simulink model "v2_2025_10_22_D1_chart_skeleton"  (R2025a)
settings: Solver=FixedStepAuto  StartTime=0.0  StopTime=10.0  FixedStep=1e-3  RelTol=1e-3  EnableMultiTasking=on
settings Model: ExtModeTrigDuration=5  Creator=zhang  LastModifiedBy=zhang
settings OptimizationCC: DefaultParameterBehavior=Inlined  EnhancedBackFolding=on  PassReuseOutputArgsAs=Individual arguments  ZeroExternalMemoryAtStartup=off  ZeroInternalMemoryAtStartup=off  MaxStackSize=64  OptimizeBlockOrder=speed  DifferentSizesBufferReuse=on  OptimizationCustomize=off  EfficientTunableParamExpr=on
settings DebuggingCC: ParameterTunabilityLossMsg=error
settings HardwareCC: ProdBitPerPointer=32.0  ProdBitPerSizeT=32.0  ProdBitPerPtrDiffT=32.0  ProdLargestAtomicInteger=Long  ProdLargestAtomicFloat=Double  ProdWordSize=32.0  ProdHWDeviceType=ARM Compatible->ARM Cortex
settings SFSimCC: MATLABDynamicMemAlloc=off
settings RTWCC: SystemTargetFile=ert.tlc  HardwareBoard=NXP FRDM-K64F  TLCOptions="-aInlineSetEventsForThisBaseRateFcn=TLC_FALSE -aSuppressMultiTaskScheduler=TLC_FALSE  -aRateBasedStepFcn=0"  TemplateMakefile=ert_default_tmf  Toolchain=GNU Tools for ARM Embedded Processors  Description=Embedded Coder
settings CodeAppCC: ForceParamTrailComments=on  IgnoreCustomStorageClasses=off  OperatorAnnotations=on  SimulinkDataObjDesc=on  SFDataObjDesc=on  InsertBlockDesc=on
settings ERTTargetCC: ExtModeTransport=4.0  ExtModeStaticAlloc=off  ExtModeMexFile=sendToCommService  ExtModeIntrfLevel=Level1

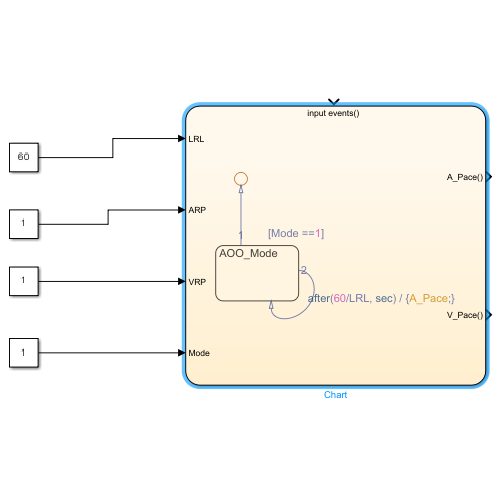
[thumbnail: Simulink's stored preview of the top-level diagram]
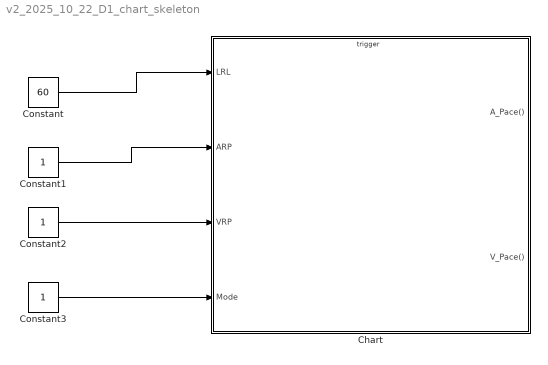
== system v2_2025_10_22_D1_chart_skeleton ==
  Chart : Stateflow chart  TreatAsAtomicUnit=on
  Constant : Constant  Value=60
  Constant1 : Constant
  Constant2 : Constant
  Constant3 : Constant
  wires:
  Constant/1 -> Chart/1(LRL)
  Constant1/1 -> Chart/2(ARP)
  Constant2/1 -> Chart/3(VRP)
  Constant3/1 -> Chart/4(Mode)

== stateflow chart v2_2025_10_22_D1_chart_skeleton/Chart ==
  state AOO_Mode
  AOO_Mode -> (junction 50) [order 1] : [Mode ==1]
  AOO_Mode -> AOO_Mode [order 2] : after(60/LRL, sec) / {A_Pace;}
  data: LRL input; ARP input; VRP input; Mode input
  events: A_Sense input FUNCTION_CALL_EVENT; V_Sense input FUNCTION_CALL_EVENT; A_Pace output FUNCTION_CALL_EVENT; V_Pace output FUNCTION_CALL_EVENT
